simulink library "rebuilt_deng_library_20261024"  (R2025a)
settings: Solver=VariableStepAuto  StartTime=0.0  StopTime=10.0  RelTol=1e-3
settings Model: Creator=Ben Bolen  LastModifiedBy=Ben Bolen

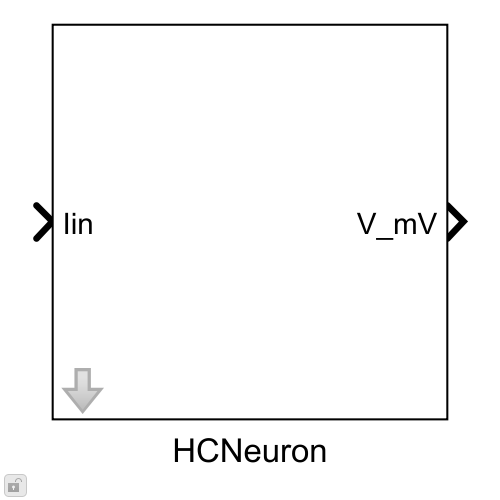
[thumbnail: Simulink's stored preview of the top-level diagram]
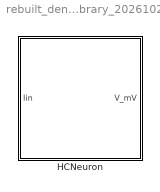
== system rebuilt_deng_library_20261024 ==
  HCNeuron : Subsystem  mask{Cm=5, Gm=1, Vrest=-60, GNa=1.5, ENa=50, Sm=0.2, Em=-40, Km=1, Sh=-0.6, Eh=-60, Kh=0.5, tauH=350, h0=0.6666667}
      mask prompts: Cm "Membrane capacitance Cm (nF)"; Gm "Membrane conductance Gm (uS)"; Vrest "Resting potential Vrest (mV)"; GNa "Persistent Na conductance GNa (uS)"; ENa "Na reversal ENa (mV)"; Sm "m-gate slope Sm"; Em "m-gate midpoint Em (mV)"; Km "m-gate constant Km"; Sh "h-gate slope Sh"; Eh "h-gate midpoint Eh (mV)"; Kh "h-gate exponent Kh"; tauH "h-gate time constant tauH (ms), FIXED"; h0 "initial h (h_inf(Vrest) = 0.6667)"
      mask help:
      | Deng/Nourse persistent-Na half-center neuron (Tables A4/A5).
      | Cm dV/dt = Gm(Vrest-V) + Iin + GNa*m*h^K*(ENa-V); m instantaneous,
      | dh/dt = (h_inf - h)/tauH with tauH FIXED (Animatlab interpretation).
      | Nourse 2023 defaults reproduce the rat hindlimb RG half-center.

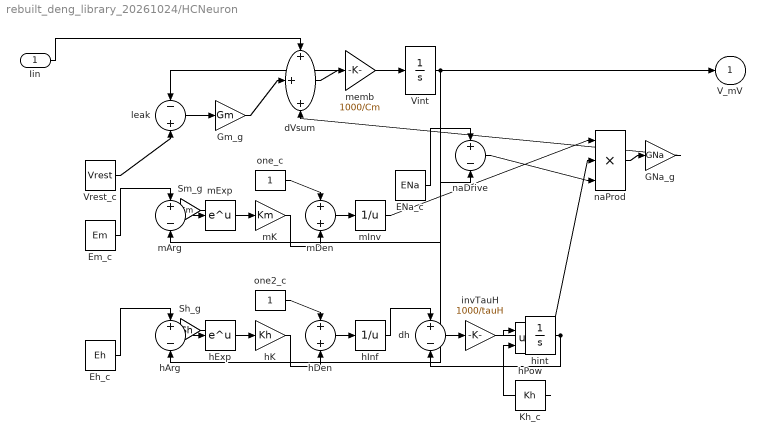
== system rebuilt_deng_library_20261024/HCNeuron ==
  Iin : Inport
  ENa_c : Constant  Value=ENa
  Eh_c : Constant  Value=Eh
  Em_c : Constant  Value=Em
  GNa_g : Gain  Gain=GNa
  Gm_g : Gain  Gain=Gm
  Kh_c : Constant  Value=Kh
  Sh_g : Gain  Gain=Sh
  Sm_g : Gain  Gain=Sm
  Vint : Integrator  InitialCondition=Vrest
  Vrest_c : Constant  Value=Vrest
  dVsum : Sum  Inputs=+++
  dh : Sum  Inputs=+-
  hArg : Sum  Inputs=+-
  hDen : Sum
  hExp : Math
  hInf : Math  Operator=reciprocal
  hK : Gain  Gain=Kh
  hPow : Math  Operator=pow
  hint : Integrator  InitialCondition=h0
  invTauH : Gain  Gain=1000/tauH
  leak : Sum  Inputs=-+
  mArg : Sum  Inputs=+-
  mDen : Sum
  mExp : Math
  mInv : Math  Operator=reciprocal
  mK : Gain  Gain=Km
  memb : Gain  Gain=1000/Cm
  naDrive : Sum  Inputs=+-
  naProd : Product  Inputs=3
  one2_c : Constant
  one_c : Constant
  V_mV : Outport
  wires:
  Iin/1 -> dVsum/1
  Vint/1 -> leak/1, V_mV/1, mArg/2, hArg/2, naDrive/2
  Vrest_c/1 -> leak/2
  leak/1 -> Gm_g/1
  Gm_g/1 -> dVsum/2
  GNa_g/1 -> dVsum/3
  dVsum/1 -> memb/1
  memb/1 -> Vint/1
  Em_c/1 -> mArg/1
  mArg/1 -> Sm_g/1
  Sm_g/1 -> mExp/1
  mExp/1 -> mK/1
  mK/1 -> mDen/2
  one_c/1 -> mDen/1
  mDen/1 -> mInv/1
  Eh_c/1 -> hArg/1
  hArg/1 -> Sh_g/1
  Sh_g/1 -> hExp/1
  hExp/1 -> hK/1
  hK/1 -> hDen/2
  one2_c/1 -> hDen/1
  hDen/1 -> hInf/1
  hInf/1 -> dh/1
  hint/1 -> dh/2, hPow/1
  dh/1 -> invTauH/1
  invTauH/1 -> hint/1
  ENa_c/1 -> naDrive/1
  mInv/1 -> naProd/1
  Kh_c/1 -> hPow/2
  hPow/1 -> naProd/2
  naDrive/1 -> naProd/3
  naProd/1 -> GNa_g/1
